simulink model "vehicle_cl"  (R2026b)
settings: Solver=FixedStepAuto  FixedStep=0.01
settings Model: DataDictionary=vehicle_control.sldd  Creator=rayyu  LastModifiedBy=bxr240009
settings RTWCC: GPUComputeCapability=5.0

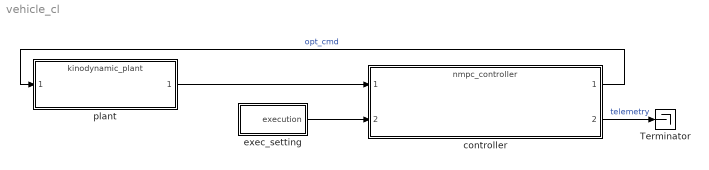
== system vehicle_cl ==
  Terminator : Terminator
  controller : ModelReference  ModelNameDialog=nmpc_controller.slx  SimulationMode=Normal  ModelReferenceVersion=3.41
  exec_setting : Subsystem
  plant : ModelReference  ModelNameDialog=kinodynamic_plant.slx  SimulationMode=Normal  ModelReferenceVersion=3.2
  wires:
  plant/1 -> controller/1
  controller/1 -> plant/1  "opt_cmd"
  exec_setting/1(execution) -> controller/2
  controller/2 -> Terminator/1  "telemetry"

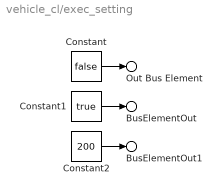
== system vehicle_cl/exec_setting ==
  Constant : Constant  Value=false  OutDataTypeStr=boolean
  Constant1 : Constant  Value=true  OutDataTypeStr=boolean
  Constant2 : Constant  Value=200
  Out Bus Element : Outport  PortName=execution  Element=reset
  BusElementOut : Outport  PortName=execution  Element=enable
  BusElementOut1 : Outport  PortName=execution  Element=cap
  wires:
  Constant/1 -> Out Bus Element/1
  Constant1/1 -> BusElementOut/1
  Constant2/1 -> BusElementOut1/1
